simulink model "sm_excv_track2"  (R2026b)
settings: Solver=ode23t  StopTime=14  FixedStep=2e-4  AbsTol=1e-3
StartFcn:
  | tic
StopFcn:
  | Elapsed_Sim_Time = toc;
  | disp(['Elapsed Sim Time = ' num2str(Elapsed_Sim_Time)]);
undefined symbols (not defined in the file): Excv, X, Y, Z
libraries: simulink x5, fl_lib x4, sm_lib x3, nesl_utility x3, sm_trackV_lib_terrain_contact x3, sm_excv_chassis_lib x2, sm_trackV_lib_chain_underc_elem x2, sm_trackV_lib_chain_lower_frame_s46i1u2l7 x2
CloseFcn:
  | try,close(h1_sm_excv_track_double),end
  | clear h1_sm_excv_track_double
  | try,close(h2_sm_excv_track_double),end
  | clear h2_sm_excv_track_double
  | try,close(h3_sm_excv_track_double),end
  | clear h3_sm_excv_track_double
  | try,close(h4_sm_excv_track_double),end
  | clear h4_sm_excv_track_double
  | 
  | 
  | clear simlog_sm_excv_track_double
  | clear logsout_sm_excv_track_double
settings Model: Creator=evo  LastModifiedBy=smiller
settings SolverCC: AutoScaleAbsTol=off
settings DataIOCC: DSMLogging=off  ReturnWorkspaceOutputs=off  SaveOutput=off  SignalLoggingName=logsout_sm_excv_track2
settings DebuggingCC: SymbolicDimsDataTypeCodeGenerationDiagnostic=none
settings SFSimCC: CustomCodeUndefinedFunction=UseInterfaceOnly
settings RTWCC: DLArmComputeVersion=19.05
settings SimscapeCC: SimscapeLogLimitData=off  SimscapeLogName=simlog_sm_excv_track2  SimscapeLogSimulationStatistics=on  SimscapeLogType=all  SimscapeUseEnergyAccounting=off
settings DiagnosticsConfigSet: SimMechanicsConflictingReferenceFrames=none
settings ExplorerConfigSet: InternalSimMechanicsExplorerSettings="<ExplorerConfiguration><canonicalview>default</canonicalview><AnimationSetting><BasePlaybackSpeed>1.0</BasePlaybackSpeed><PlaybackSpeedFactor>2.0</PlaybackSpeedFactor></AnimationSetting><TilePanel><TileInfo><Tiles Columns=\"2\" Count=\"3\" Rows=\"2\"><Column Weight=\"0.5\"/><Column Weight=\"0.5\"/><Row Weight=\"0.4992\"/><Row Weight=\"0.5008\"/><Tile Height=\"1\" Width=\"2\" X=\"0\" Y=\"0\"/><Tile Height=\"1\" Width=\"1\" X=\"0\" Y=\"1\"/><Tile Height=\"1\" Width=\"1\" X=\"1\" Y=\"1\"/></Tiles></TileInfo><SceneInfo><SceneViewer><BGColor><R>1</R><G>1</G><B>1</B></BGColor><Camera><DoPerspective>on</DoPerspective><Position><X>-0.142135607180110757</X><Y>-0.0627421547287057291</Y><Z>-0.0901753349307433949</Z></Position><Center><X>0.857864392819889243</X><Y>-0.0627421547287057291</Y><Z>-0.0901753349307433949</Z></Center><Up><X>0</X><Y>0</Y><Z>1</Z></Up><ViewLimDist>1</ViewLimDist><YLim>0.466307658154998583</YLim><XLim>2.00735865171518224</XLim></Camera></SceneViewer><SceneViewer><BGColor><R>1</R><G>1</G><B>1</B></BGColor><Camera><DoPerspective>on</DoPerspective><Position><X>5.3724028067841374</X><Y>-4.14362388366202694</Y><Z>3.11224490535173137</Z></Position><Center><X>1.53829089639127714</X><Y>-0.0431681887141522891</Y><Z>0.0323343624376755678</Z></Center><Up><X>0</X><Y>0</Y><Z>1</Z></Up><ViewLimDist>1</ViewLimDist><YLim>0.466307658154998583</YLim><XLim>0.996493077701092966</XLim></Camera></SceneViewer><SceneViewer><BGColor><R>1</R><G>1</G><B>1</B></BGColor><Camera><DoPerspective>on</DoPerspective><Position><X>1.59934586807766643</X><Y>-4.0377364579651962</Y><Z>-0.166905775900695108</Z></Position><Center><X>1.58408212515606928</X><Y>-3.03909439065243525</Y><Z>-0.117095741316102439</Z></Center><Up><X>0</X><Y>0</Y><Z>1</Z></Up><ViewLimDist>1</ViewLimDist><YLim>0.466307658154998583</YLim><XLim>0.996493077701092966</XLim></Camera></SceneViewer></SceneInfo></TilePanel><MechEditorPanel><Cameras><Camera><Id>Camera1</Id><Value><Name>Track_CtrRear_AimFront</Name><NativeCamera><PositionTrackingFeature>Chassis.Camera_Frames.CamF_CtrRear_AimLF.R</PositionTrackingFeature><CenterTrackingFeature>Config.World_Frame.W</CenterTrackingFeature><UpVectorTrackingFeature>Config.World_Frame.W</UpVectorTrackingFeature><CenterTrackingOrigin>off</CenterTrackingOrigin><CenterTrackingDirection>+X</CenterTrackingDirection><UpVectorTrackingDirection>+Z</UpVectorTrackingDirection></NativeCamera></Value></Camera><Camera><Id>Camera2</Id><Value><Name>Track_Left_AimRight</Name><NativeCamera><PositionTrackingFeature>Chassis.Camera_Frames.CamF_Left_AimRight.R</PositionTrackingFeature><CenterTrackingFeature>Chassis.Camera_Frames.CamF_Left_AimRight.R</CenterTrackingFeature><UpVectorTrackingFeature>Config.World_Frame.W</UpVectorTrackingFeature><CenterTrackingOrigin>off</CenterTrackingOrigin><CenterTrackingDirection>+X</CenterTrackingDirection><UpVectorTrackingDirection>+Z</UpVectorTrackingDirection></NativeCamera></Value></Camera><Camera><Id>Camera3</Id><Value><Name>Track_Front_AimLR</Name><NativeCamera><PositionTrackingFeature>Chassis.Camera_Frames.CamF_Front_AimLR.R</PositionTrackingFeature><CenterTrackingFeature>Chassis.Camera_Frames.Transform_Aim_LR.F</CenterTrackingFeature><UpVectorTrackingFeature>Config.World_Frame.W</UpVectorTrackingFeature><CenterTrackingOrigin>off</CenterTrackingOrigin><CenterTrackingDirection>+X</CenterTrackingDirection><UpVectorTrackingDirection>+Z</UpVectorTrackingDirection></NativeCamera></Value></Camera><Camera><Id>Camera4</Id><Value><Name>Track_Right_AimLeftTL</Name><NativeCamera><PositionTrackingFeature>Chassis.Camera_Frames.CamF_Right_AimLeftTL.R</PositionTrackingFeature><CenterTrackingFeature>Chassis.Camera_Frames.CamF_Right_AimLeftTL.R</CenterTrackingFeature><UpVectorTrackingFeature>Config.World_Frame.W</UpVectorTrackingFeature><CenterTrackingOrigin>off</CenterTrackingOrigin><CenterTrackingDirection>+X</CenterTrackingDirection><UpVectorTrackingDirection>+Z</UpVectorTrackingDirection></NativeCamera></Value></Camera><Camera><Id>Camera5</Id><Value><Name>Track_Right_AimLeftTR</Name><NativeCamera><PositionTrackingFeature>Chassis.Camera_Frames.CamF_Right_AimLeftTR.R</PositionTrackingFeature><CenterTrackingFeature>Chassis.Camera_Frames.CamF_Right_AimLeftTR.R</CenterTrackingFeature><UpVectorTrackingFeature>Config.World_Frame.W</UpVectorTrackingFeature><CenterTrackingOrigin>off</CenterTrackingOrigin><CenterTrackingDirection>+X</CenterTrackingDirection><UpVectorTrackingDirection>+Z</UpVectorTrackingDirection></NativeCamera></Value></Camera><Camera><Id>Camera6</Id><Value><Name>Track_FR_AimFront</Name><NativeCamera><PositionTrackingFeature>Chassis.Camera_Frames.CamF_FR_Aim_Front_R</PositionTrackingFeature><CenterTrackingFeature>Chassis.Camera_Frames.CamF_FR_Aim_Front_R</CenterTrackingFeature><UpVectorTrackingFeature>Config.W</UpVectorTrackingFeature><CenterTrackingOrigin>off</CenterTrackingOrigin><CenterTrackingDirection>+X</CenterTrackingDirection><UpVectorTrackingDirection>+Z</UpVectorTrackingDirection></NativeCamera></Value></Camera><Camera><Id>Camera7</Id><Value><Name>Track_FR_AimCtr</Name><NativeCamera><PositionTrackingFeature>Chassis.Camera_Frames.CamF_FR_AimCtr.R</PositionTrackingFeature><CenterTrackingFeature>Chassis.Camera_Frames.Transform_Ctr.F</CenterTrackingFeature><UpVectorTrackingFeature>Config.World_Frame.W</UpVectorTrackingFeature><CenterTrackingOrigin>on</CenterTrackingOrigin><UpVectorTrackingDirection>+Z</UpVectorTrackingDirection></NativeCamera></Value></Camera></Cameras><GfxPanelCameraMap><MapElement CameraMLId=\"Camera1\" GfxPanelIndex=\"0\"/><MapElement CameraMLId=\"Camera7\" GfxPanelIndex=\"1\"/><MapElement CameraMLId=\"Camera5\" GfxPanelIndex=\"2\"/></GfxPanelCameraMap><VideoCreator><PlaybackSpeedRatio>1.0</PlaybackSpeedRatio><FrameRate>30</FrameRate><VideoFormat>Motion JPEG AVI</VideoFormat><FrameSize>auto</FrameSize></VideoCreator></MechEditorPanel></ExplorerConfiguration>"

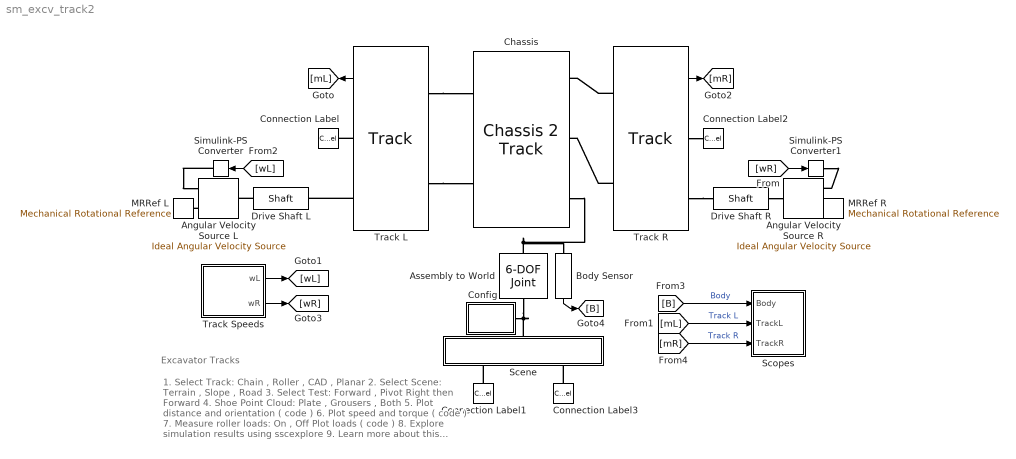
== system sm_excv_track2 ==
  note: Excavator Tracks
  note: 1. Select Track: Chain , Roller , CAD , Planar
      | 2. Select Scene: Terrain , Slope , Road
      | 3. Select Test: Forward , Pivot Right then Forward
      | 4. Shoe Point Cloud: Plate , Grousers , Both
      | 5. Plot distance and orientation ( code )
      | 6. Plot speed and torque ( code )
      | 7. Measure roller loads: On , Off Plot loads ( code )
      | 8. Explore simulation results using sscexplore
      | 9. Learn more about this example
  Angular Velocity Source L : fl_lib/Mechanical/Mechanical Sources/Ideal Angular Velocity Source
  Angular Velocity Source R : fl_lib/Mechanical/Mechanical Sources/Ideal Angular Velocity Source
  Assembly to World : sm_lib/Joints/6-DOF Joint  JointMode=Normal  CompositeWrenchDir=FollowerOnBase  CompositeWrenchFrame=BaseFrame  SenseConstraintForce=off  SenseConstraintTorque=off  SenseTotalForce=off  SenseTotalTorque=off  PxPositionTargetSpecify=on  PxPositionTargetPriority=High  PxPositionTargetValue=0  PxPositionTargetValueUnits=m  PxVelocityTargetSpecify=off  PxVelocityTargetPriority=High  PxVelocityTargetValue=0  PxVelocityTargetValueUnits=m/s  PxEquilibriumPosition=0  PxEquilibriumPositionUnits=m  PxSpringStiffness=0  PxSpringStiffnessUnits=N/m  PxDampingCoefficient=0  PxDampingCoefficientUnits=N/(m/s)  PxLowerLimitSpecify=off  PxLowerLimitBound=-1  PxLowerLimitBoundUnits=m  PxLowerLimitStiffness=1e6  PxLowerLimitStiffnessUnits=N/m  PxLowerLimitDamping=1e3  PxLowerLimitDampingUnits=N/(m/s)  PxLowerLimitTransitionRegionWidth=1e-4  PxLowerLimitTransitionRegionWidthUnits=m  PxUpperLimitSpecify=off  PxUpperLimitBound=1  PxUpperLimitBoundUnits=m  PxUpperLimitStiffness=1e6  PxUpperLimitStiffnessUnits=N/m  PxUpperLimitDamping=1e3  PxUpperLimitDampingUnits=N/(m/s)  PxUpperLimitTransitionRegionWidth=1e-4  PxUpperLimitTransitionRegionWidthUnits=m  PxTorqueActuationMode=NoTorque  PxMotionActuationMode=ComputedMotion  PxSensePosition=off  PxSenseVelocity=off  PxSenseAcceleration=off  PxSenseTorqueForce=off  PxSenseLowerLimitTorqueForce=off  PxSenseUpperLimitTorqueForce=off  PyPositionTargetSpecify=on  PyPositionTargetPriority=High  PyPositionTargetValue=0  PyPositionTargetValueUnits=m  PyVelocityTargetSpecify=off  PyVelocityTargetPriority=High  PyVelocityTargetValue=0  PyVelocityTargetValueUnits=m/s  PyEquilibriumPosition=0  PyEquilibriumPositionUnits=m  PySpringStiffness=0  PySpringStiffnessUnits=N/m  PyDampingCoefficient=0  PyDampingCoefficientUnits=N/(m/s)  PyLowerLimitSpecify=off  PyLowerLimitBound=-1  PyLowerLimitBoundUnits=m  PyLowerLimitStiffness=1e6  PyLowerLimitStiffnessUnits=N/m  PyLowerLimitDamping=1e3  PyLowerLimitDampingUnits=N/(m/s)  PyLowerLimitTransitionRegionWidth=1e-4  PyLowerLimitTransitionRegionWidthUnits=m  PyUpperLimitSpecify=off  PyUpperLimitBound=1  PyUpperLimitBoundUnits=m  PyUpperLimitStiffness=1e6  PyUpperLimitStiffnessUnits=N/m  PyUpperLimitDamping=1e3  PyUpperLimitDampingUnits=N/(m/s)  PyUpperLimitTransitionRegionWidth=1e-4  PyUpperLimitTransitionRegionWidthUnits=m  PyTorqueActuationMode=NoTorque  PyMotionActuationMode=ComputedMotion  PySensePosition=off  PySenseVelocity=off  PySenseAcceleration=off  PySenseTorqueForce=off  PySenseLowerLimitTorqueForce=off  PySenseUpperLimitTorqueForce=off  PzPositionTargetSpecify=on  PzPositionTargetPriority=High  PzPositionTargetValue=Excv.Sprocket.sprocket_rPitch+0.2  PzPositionTargetValueUnits=m  PzVelocityTargetSpecify=off  PzVelocityTargetPriority=High  PzVelocityTargetValue=0  PzVelocityTargetValueUnits=m/s  PzEquilibriumPosition=0  PzEquilibriumPositionUnits=m  PzSpringStiffness=0  PzSpringStiffnessUnits=N/m  PzDampingCoefficient=0  PzDampingCoefficientUnits=N/(m/s)  PzLowerLimitSpecify=off  PzLowerLimitBound=-1  PzLowerLimitBoundUnits=m  PzLowerLimitStiffness=1e6  PzLowerLimitStiffnessUnits=N/m  PzLowerLimitDamping=1e3  PzLowerLimitDampingUnits=N/(m/s)  PzLowerLimitTransitionRegionWidth=1e-4  PzLowerLimitTransitionRegionWidthUnits=m  PzUpperLimitSpecify=off  PzUpperLimitBound=1  PzUpperLimitBoundUnits=m  PzUpperLimitStiffness=1e6  PzUpperLimitStiffnessUnits=N/m  PzUpperLimitDamping=1e3  PzUpperLimitDampingUnits=N/(m/s)  PzUpperLimitTransitionRegionWidth=1e-4  PzUpperLimitTransitionRegionWidthUnits=m  PzTorqueActuationMode=NoTorque  PzMotionActuationMode=ComputedMotion  PzSensePosition=off  PzSenseVelocity=off  PzSenseAcceleration=off  PzSenseTorqueForce=off  PzSenseLowerLimitTorqueForce=off  PzSenseUpperLimitTorqueForce=off  SphPositionTargetSpecify=off  SphPositionTargetPriority=High  SphPositionTargetRotationMethod=StandardAxis  SphPositionTargetFollAlignAxisA=+X  SphPositionTargetBaseAlignAxisA=+Y  SphPositionTargetFollAlignAxisB=+Y  SphPositionTargetBaseAlignAxisB=+Z  SphPositionTargetRotationStandardAxis=+Z  SphPositionTargetRotationAngle=180  SphPositionTargetRotationAngleUnits=deg  SphPositionTargetRotationArbitraryAxis=[0 0 1]  SphPositionTargetRotationSequenceAxes=FollowerAxes  SphPositionTargetRotationSequence=XYX  SphPositionTargetRotationSequenceAngles=[0 0 0]  SphPositionTargetRotationSequenceAnglesUnits=deg  SphPositionTargetRotationMatrix=[1 0 0; 0 1 0; 0 0 1]  SphPositionTargetQuaternion=[1 0 0 0]  SphVelocityTargetSpecify=off  SphVelocityTargetPriority=High  SphVelocityTargetValue=[0 0 0]  SphVelocityTargetValueUnits=deg/s  SphVelocityTargetInFollowerFrame=on  SphEqPosRotationMethod=None  SphEqPosFollAlignAxisA=+X  SphEqPosBaseAlignAxisA=+Y  SphEqPosFollAlignAxisB=+Y  SphEqPosBaseAlignAxisB=+Z  SphEqPosRotationStandardAxis=+Z  SphEqPosRotationAngle=0.0  SphEqPosRotationAngleUnits=deg  SphEqPosRotationArbitraryAxis=[0 0 1]  SphEqPosRotationSequenceAxes=FollowerAxes  SphEqPosRotationSequence=XYX  SphEqPosRotationSequenceAngles=[0 0 0]  SphEqPosRotationSequenceAnglesUnits=deg  SphEqPosRotationMatrix=[1 0 0; 0 1 0; 0 0 1]  SphEqPosQuaternion=[1 0 0 0]  SphSpringStiffness=0  SphSpringStiffnessUnits=N*m/deg  SphDampingCoefficient=0  SphDampingCoefficientUnits=N*m/(deg/s)  SphLowerLimitSpecify=off  SphLowerLimitBound=15  SphLowerLimitBoundUnits=deg  SphLowerLimitStiffness=1e4  SphLowerLimitStiffnessUnits=N*m/deg  SphLowerLimitDamping=10  SphLowerLimitDampingUnits=N*m/(deg/s)  SphLowerLimitTransitionRegionWidth=0.1  SphLowerLimitTransitionRegionWidthUnits=deg  SphUpperLimitSpecify=off  SphUpperLimitBound=45  SphUpperLimitBoundUnits=deg  SphUpperLimitStiffness=1e4  SphUpperLimitStiffnessUnits=N*m/deg  SphUpperLimitDamping=10  SphUpperLimitDampingUnits=N*m/(deg/s)  SphUpperLimitTransitionRegionWidth=0.1  SphUpperLimitTransitionRegionWidthUnits=deg  SphTorqueActuationMode=NoTorque  SphActuateTorqueX=off  SphActuateTorqueY=off  SphActuateTorqueZ=off  SphActuateTorque=off  SphActuationFrame=BaseFrame  SphSensePosition=off  SphSenseVelocityX=off  SphSenseVelocityY=off  SphSenseVelocityZ=off  SphSenseVelocity=off  SphSenseAccelerationX=off  SphSenseAccelerationY=off  SphSenseAccelerationZ=off  SphSenseAcceleration=off  SphSenseLowerLimitTorqueMag=off  SphSenseUpperLimitTorqueMag=off  SphSensingFrame=BaseFrame
  Body Sensor : sm_excv_chassis_lib/Body Sensor  offset_body_sensor=[0 0 0]
  Chassis : sm_excv_chassis_lib/Chassis 2 Track  offset_cg=Excv.Chassis.CGOffset  offset_axle=Excv.Chassis.AxleOffset  offset_Lcyl=Excv.Chassis.SuspOffset  offset_sprk2axle_x=Excv.Frame.AxleX  offset_sprk2axle_y=Excv.Frame.AxleY  Camera=Excv.Chassis.Camera  track_sep_ctr=Excv.Chassis.TrackSepCtr  axle_rad=Excv.Chassis.AxleRad  axle_opc=0  chassis_mass=Excv.Chassis.Mass  chassis_moi=Excv.Chassis.MOI  chassis_poi=Excv.Chassis.POI  body_clr=[1 1 0]  trim_clr=[0.4 0.4 0.4]  accent_clr=[1 0.6 0]  chassis_opc=1  cyl_len=Excv.Chassis.Susp.Cylinder.Cylinder.Len  cyl_rad=Excv.Chassis.Susp.Cylinder.Cylinder.Rad  cyl_mass=Excv.Chassis.Susp.Cylinder.Cylinder.Mass  piston_len=Excv.Chassis.Susp.Cylinder.Piston.Len  piston_rad=Excv.Chassis.Susp.Cylinder.Piston.Rad  piston_mass=Excv.Chassis.Susp.Cylinder.Piston.Mass  spr_k=Excv.Chassis.Susp.Cylinder.k  spr_d=Excv.Chassis.Susp.Cylinder.b  spr_xeq=Excv.Chassis.Susp.Cylinder.xeq
  Config : Subsystem
  Connection Label : ConnectionLabel  Label=GL
  Connection Label1 : ConnectionLabel  Label=GL
  Connection Label2 : ConnectionLabel  Label=GR
  Connection Label3 : ConnectionLabel  Label=GR
  Drive Shaft L : sm_trackV_lib_chain_underc_elem/Shaft  k_shaft=Excv.Drive.Shaft.k  b_shaft=Excv.Drive.Shaft.b
  Drive Shaft R : sm_trackV_lib_chain_underc_elem/Shaft  k_shaft=Excv.Drive.Shaft.k  b_shaft=Excv.Drive.Shaft.b
  MRRef L : fl_lib/Mechanical/Rotational Elements/Mechanical Rotational Reference
  MRRef R : fl_lib/Mechanical/Rotational Elements/Mechanical Rotational Reference
  Scene : Subsystem  Variant=on  VariantControlMode=label  LabelModeActiveChoice=Terrain
      settings: AttributesFormatString=%<LabelModeActiveChoice>
      mask Display: disp(' ');
  Scopes : Subsystem
  Simulink-PS Converter : nesl_utility/Simulink-PS Converter  PhysicalDomain=network_engine_domain  SubClassName=ps_input  LeftPortType=input  RightPortType=output  PseudoPeriodic=off  Frequencies=[]  NoiseDistribution=none  NoiseParameters=[]  Unit=1  AffineConversion=off  FilteringAndDerivatives=provide  SimscapeFilterOrder=1  InputFilterTimeConstant=0.001  UdotUserProvided=0
  Simulink-PS Converter1 : nesl_utility/Simulink-PS Converter  PhysicalDomain=network_engine_domain  SubClassName=ps_input  LeftPortType=input  RightPortType=output  PseudoPeriodic=off  Frequencies=[]  NoiseDistribution=none  NoiseParameters=[]  Unit=1  AffineConversion=off  FilteringAndDerivatives=provide  SimscapeFilterOrder=1  InputFilterTimeConstant=0.001  UdotUserProvided=0
  Track L : sm_trackV_lib_chain_lower_frame_s46i1u2l7/Track  LabelModeActiveChoice=ChainPts  popup_trackModel=Chain, Points  popup_leftOrRight=Left  popup_sense_roller=Actuator Torque
      settings: AttributesFormatString=|
      | %<popup_trackModel>
      | %<popup_sense_roller>
  Track R : sm_trackV_lib_chain_lower_frame_s46i1u2l7/Track  LabelModeActiveChoice=ChainPts  popup_trackModel=Chain, Points  popup_leftOrRight=Right  popup_sense_roller=Actuator Torque
      settings: AttributesFormatString=|
      | %<popup_trackModel>
      | %<popup_sense_roller>
  Track Speeds : Subsystem  Variant=on  VariantControlMode=label  VariantControl=Choice  LabelModeActiveChoice=Fwd
      settings: AttributesFormatString=%<LabelModeActiveChoice>
      mask Display: disp(' ')
  wires:
  Track L/1 -> [mL]
  [mL] -> Scopes/2(TrackL)  "Track L"
  Track R/1 -> [mR]
  [mR] -> Scopes/3(TrackR)  "Track R"
  Track Speeds/1(wL) -> [wL]
  [wL] -> Simulink-PS Converter/1
  Track Speeds/2(wR) -> [wR]
  [wR] -> Simulink-PS Converter1/1
  Body Sensor/1 -> [B]
  [B] -> Scopes/1(Body)  "Body"
  connections:
  Assembly to World/LConn1 -- Scene/RConn1 -- Config/LConn1
  Assembly to World/RConn1 -- Body Sensor/LConn1 -- Chassis/RConn3
  Drive Shaft L/LConn1 -- Angular Velocity Source L/LConn1
  Simulink-PS Converter/RConn1 -- Angular Velocity Source L/RConn1
  Angular Velocity Source L/RConn2 -- MRRef L/LConn1
  Angular Velocity Source R/RConn2 -- MRRef R/LConn1
  Simulink-PS Converter1/RConn1 -- Angular Velocity Source R/RConn1
  Drive Shaft R/LConn1 -- Angular Velocity Source R/LConn1
  Track L/LConn1 -- Chassis/LConn1
  Track L/LConn2 -- Chassis/LConn2
  Track L/RConn2 -- Drive Shaft L/RConn1
  Track R/LConn1 -- Chassis/RConn1
  Track R/LConn2 -- Chassis/RConn2
  Track R/RConn2 -- Drive Shaft R/RConn1
  Track L/RConn1 -- Connection Label/LConn1
  Track R/RConn1 -- Connection Label2/LConn1
  Connection Label1/LConn1 -- Scene/LConn1
  Connection Label3/LConn1 -- Scene/LConn2

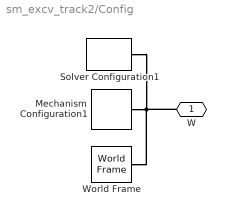
== system sm_excv_track2/Config ==
  Mechanism Configuration1 : sm_lib/Utilities/Mechanism Configuration  UniformGravity=Constant  GravityVector=[0 0 -9.80665]  GravityVectorUnits=m/s^2  LinearizationDelta=0.001  JointModeTransitionNonlinearIterations=2
  Solver Configuration1 : nesl_utility/Solver Configuration  PhysicalDomain=network_engine_domain  SubClassName=solver  LeftPortType=input  RightPortType=generic  Tones=[]  Harmonics=[]  SimulateNoise=off  Profile=off  UseLocalSampling=off  EnableSwitchedLinearOptims=on  FrequencyDomain=off  UseCCode=off  RelTol=0.001  AbsTol=0.001  MinStep=1e-09  ToWorkspace=off  RevertToSquareIcSolve=off  NumHomotopyIterations=100  PhasorMode=off  PhasorModeNumHarmonics=1  ConsistencySolver=NEWTON_FTOL  CanonicalOrdering=UNORDERED  OptimizeIntermediates=UNOPTIMIZED  MulticoreSolverChoice=BACKWARD_EULER  IndexReductionMethod=DerivativeReplacement  DoDC=off  ResidualTolerance=1e-09  ConsistencyTolSource=GLOBAL  ConsistencyAbsTol=0.001  ConsistencyRelTol=0.001  ConsistencyTolFactor=0.001  UseLocalSolver=off  LocalSolverChoice=NE_BACKWARD_EULER_ADVANCER  ResolveIndetEquations=on  FunctionEvalNumThread=1  LocalSolverSampleTime=0.001  DoFixedCost=off  MaxNonlinIter=3  MaxModeIter=2  ComputeImpulses=off  ImpulseIterations=2  LinearAlgebra=auto  LinearAlgebraNumThread=0  EquationFormulation=NE_TIME_EF  DelaysMemoryBudget=1024  AutomaticFiltering=on  FilteringTimeConstant=0.001  PartitionStorageMethod=AS_NEEDED  PartitionMemoryBudget=1024  PartitionMethod=BALANCED  MultibodyUseLocalSolver=off  MultibodyLocalSolverChoice=ODE1  MultibodyLocalSolverSampleTime=0.001
  World Frame : sm_lib/Frames and Transforms/World Frame
  W : PMIOPort  Side=Left
  connections:
  W/RConn1 -- Solver Configuration1/RConn1 -- Mechanism Configuration1/RConn1 -- World Frame/RConn1

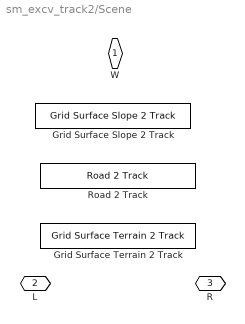
== system sm_excv_track2/Scene ==
  Grid Surface Slope 2 Track : sm_trackV_lib_terrain_contact/Grid Surface Slope 2 Track  VariantControl=Slope  road_len=Scene.Slope.road_len  road_wid=Scene.Slope.road_wid  slope_rise=Scene.Slope.slope_rise  slope_run=Scene.Slope.slope_run  slope_x0=Scene.Slope.slope_start  slope_xres=Scene.Slope.slope_xres  surface_clr=Scene.Slope.clr  surface_opc=Scene.Slope.opc  TW_Road=Scene.Contact.Terrain.TW  B_Road=Scene.Contact.Terrain.B  K_Road=Scene.Contact.Terrain.K  F_dyn_Road=Scene.Contact.Terrain.mud  F_stat_Road=Scene.Contact.Terrain.mus  CV_Road=Scene.Contact.Terrain.CV
  Grid Surface Terrain 2 Track : sm_trackV_lib_terrain_contact/Grid Surface Terrain 2 Track  SystemSampleTime=-1  VariantControl=Terrain  VariantActivationTime=update diagram  EmptyChoice=off  PassThrough=off  PassThroughVariantControl=(default)  EmptyChoiceVariantControl=(default)  AllowFlexibleInterface=on  Latency=0  AutoFrameSizeCalculation=off
  Road 2 Track : sm_trackV_lib_terrain_contact/Road 2 Track  SystemSampleTime=-1  VariantControl=Road  VariantActivationTime=update diagram  EmptyChoice=off  PassThrough=off  PassThroughVariantControl=(default)  EmptyChoiceVariantControl=(default)  AllowFlexibleInterface=on  Latency=0  AutoFrameSizeCalculation=off
  W : PMIOPort  Side=Right
  L : PMIOPort  Port=2  Side=Left
  R : PMIOPort  Port=3  Side=Left

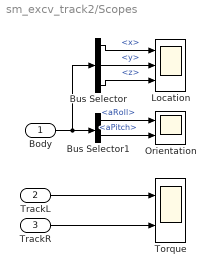
== system sm_excv_track2/Scopes ==
  Body : Inport
  TrackL : Inport  Port=2
  TrackR : Inport  Port=3
  Bus Selector : BusSelector  OutputSignals=x,y,z
  Bus Selector1 : BusSelector  OutputSignals=aRoll,aPitch
  Location : Scope  NumInputPorts=3
      settings: ActiveDisplayYMinimum=-2.438  ActiveDisplayYMaximum=13.72233
  Orientation : Scope  NumInputPorts=2
      settings: ActiveDisplayYMinimum=-0.40552  ActiveDisplayYMaximum=0.36121  DataLoggingVariableName=ScopeData2
  Torque : Scope  NumInputPorts=2
  wires:
  Body/1 -> Bus Selector/1, Bus Selector1/1
  Bus Selector/3 -> Location/3  "<z>"
  TrackL/1 -> Torque/1
  Bus Selector1/1 -> Orientation/1  "<aRoll>"
  Bus Selector/2 -> Location/2  "<y>"
  Bus Selector/1 -> Location/1  "<x>"
  Bus Selector1/2 -> Orientation/2  "<aPitch>"
  TrackR/1 -> Torque/2

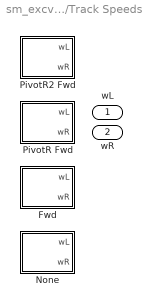
== system sm_excv_track2/Track Speeds ==
  Fwd : Subsystem  VariantControl=Fwd
  None : Subsystem  VariantControl=None
  PivotR Fwd : Subsystem  VariantControl=PivotR_Fwd
  PivotR2 Fwd : Subsystem  VariantControl=PivotR2_Fwd
  wL : Outport
  wR : Outport  Port=2

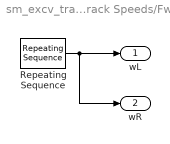
== system sm_excv_track2/Track Speeds/Fwd ==
  Repeating Sequence : simulink/Sources/Repeating Sequence  rep_seq_t=[0 2 2.01 40]  rep_seq_y=[0 0 3 3]
  wL : Outport
  wR : Outport  Port=2
  wires:
  Repeating Sequence/1 -> wR/1, wL/1

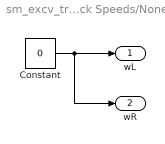
== system sm_excv_track2/Track Speeds/None ==
  Constant : Constant  Value=0
  wL : Outport
  wR : Outport  Port=2
  wires:
  Constant/1 -> wL/1, wR/1

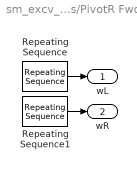
== system sm_excv_track2/Track Speeds/PivotR Fwd ==
  Repeating Sequence : simulink/Sources/Repeating Sequence  rep_seq_t=[0 2 2.01 40]  rep_seq_y=[0 0 3 3]
  Repeating Sequence1 : simulink/Sources/Repeating Sequence  rep_seq_t=[0 2 2.01 2.5 2.51 40]  rep_seq_y=[0 0 -3 -3 3 3]
  wL : Outport
  wR : Outport  Port=2
  wires:
  Repeating Sequence1/1 -> wR/1
  Repeating Sequence/1 -> wL/1

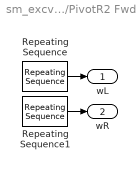
== system sm_excv_track2/Track Speeds/PivotR2 Fwd ==
  Repeating Sequence : simulink/Sources/Repeating Sequence  rep_seq_t=[0 2 2.01 40]  rep_seq_y=[0 0 3 3]
  Repeating Sequence1 : simulink/Sources/Repeating Sequence  rep_seq_t=[0 2 2.01 5.5 5.51 40]  rep_seq_y=[0 0 -3 -3 3 3]
  wL : Outport
  wR : Outport  Port=2
  wires:
  Repeating Sequence/1 -> wL/1
  Repeating Sequence1/1 -> wR/1
